simulink model "contrPUMA"  (R2026b)
settings: Solver=ode45  StopTime=7  MaxStep=1e-2  RelTol=1e-6  AbsTol=1e-8
libraries: slpidlib x3
settings Model: Creator=horia  LastModifiedBy=horia
settings DebuggingCC: AlgebraicLoopMsg=none

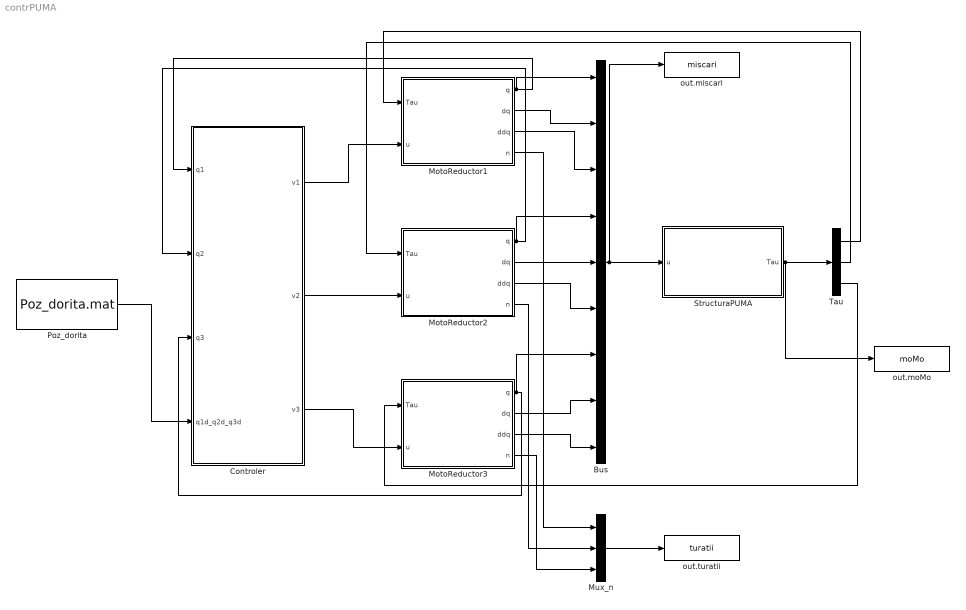
== system contrPUMA ==
  Bus : Mux  Inputs=9
  Controler : Subsystem
  MotoReductor1 : Subsystem
      settings: AttributesFormatString=RE 40 148867 + GP 52 C 230:1 (223101)
  MotoReductor2 : Subsystem
      settings: AttributesFormatString=RE 40 148867 + GP 52 C 230:1 (223101)
  MotoReductor3 : Subsystem
      settings: AttributesFormatString=RE 40 148867 + GP 42 C 74:1 (203123)
  Mux_n : Mux  Inputs=3
  Poz_dorita : FromFile  FileName=Poz_dorita.mat  SampleTime=0  ExtrapolationBeforeFirstDataPoint=Hold first value  ExtrapolationAfterLastDataPoint=Hold last value
  StructuraPUMA : Subsystem
  Tau : Demux  Outputs=3
  out.miscari : ToWorkspace  VariableName=miscari  SaveFormat=Timeseries  SampleTime=-1
  out.moMo : ToWorkspace  VariableName=moMo  SaveFormat=Timeseries  SampleTime=-1
  out.turatii : ToWorkspace  VariableName=turatii  SaveFormat=Timeseries  SampleTime=-1
  wires:
  Poz_dorita/1 -> Controler/4(q1d_q2d_q3d)
  Controler/1(v1) -> MotoReductor1/2(u)
  MotoReductor1/1(q) -> Controler/1(q1), Bus/1
  MotoReductor1/2(dq) -> Bus/2
  MotoReductor1/3(ddq) -> Bus/3
  MotoReductor1/4(n) -> Mux_n/1
  Tau/1 -> MotoReductor1/1(Tau)
  Controler/2(v2) -> MotoReductor2/2(u)
  MotoReductor2/1(q) -> Controler/2(q2), Bus/4
  MotoReductor2/2(dq) -> Bus/5
  MotoReductor2/3(ddq) -> Bus/6
  MotoReductor2/4(n) -> Mux_n/2
  Tau/2 -> MotoReductor2/1(Tau)
  Controler/3(v3) -> MotoReductor3/2(u)
  MotoReductor3/1(q) -> Controler/3(q3), Bus/7
  MotoReductor3/2(dq) -> Bus/8
  MotoReductor3/3(ddq) -> Bus/9
  MotoReductor3/4(n) -> Mux_n/3
  Tau/3 -> MotoReductor3/1(Tau)
  Bus/1 -> StructuraPUMA/1(u), out.miscari/1
  StructuraPUMA/1(Tau) -> Tau/1, out.moMo/1
  Mux_n/1 -> out.turatii/1

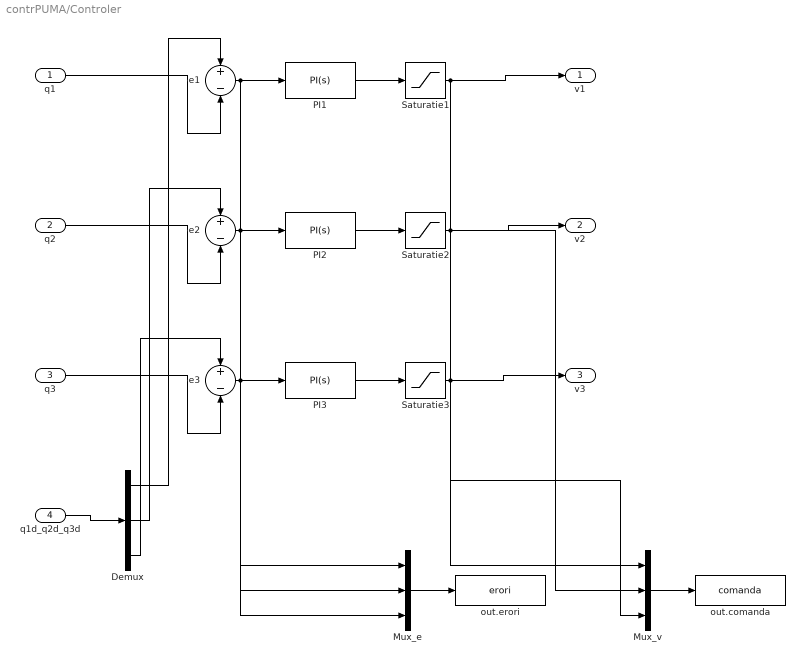
== system contrPUMA/Controler ==
  q1 : Inport  PortDimensions=1
  q2 : Inport  Port=2  PortDimensions=1
  q3 : Inport  Port=3  PortDimensions=1
  q1d_q2d_q3d : Inport  Port=4  PortDimensions=3
  Demux : Demux  Outputs=3
  Mux_e : Mux  Inputs=3
  Mux_v : Mux  Inputs=3
  PI1 : slpidlib/PID Controller  Controller=PI  Form=Parallel  TimeDomain=Continuous-time  UseExternalTs=off  SampleTime=-1  IntegratorMethod=Forward Euler  FilterMethod=Forward Euler  ControllerParametersSource=internal  P=108.8336797  I=567.4519736  UseKiTs=off  D=0  UseExternalDerivativeSource=off  N=100  UseFilter=on  TunerSelectOption=Transfer Function Based (PID Tuner App)  InitialConditionSource=internal  InitialConditionForIntegrator=0  InitialConditionForFilter=0  DifferentiatorICPrevScaledInput=0  ExternalReset=none  TrackingMode=off  Kt=1  LimitOutput=off  SatLimitsSource=internal  UpperSaturationLimit=inf  LowerSaturationLimit=-inf  LinearizeAsGain=on  AntiWindupMode=none  Kb=1  LimitIntegrator=off  UpperIntegratorSaturationLimit=inf  LowerIntegratorSaturationLimit=-inf  POutMin=[]  POutMax=[]  IOutMin=[]  IOutMax=[]  DOutMin=[]  DOutMax=[]  NOutMin=[]  NOutMax=[]  SumOutMin=[]  SumOutMax=[]  SaturationOutMin=[]  SaturationOutMax=[]  PParamMin=[]  PParamMax=[]  IParamMin=[]  IParamMax=[]  DParamMin=[]  DParamMax=[]  NParamMin=[]  NParamMax=[]  KbParamMin=[]  KbParamMax=[]  KtParamMin=[]  KtParamMax=[]  KbOutMin=[]  KbOutMax=[]  KtOutMin=[]  KtOutMax=[]  IntegratorOutMin=[]  IntegratorOutMax=[]  FilterOutMin=[]  FilterOutMax=[]  SumI1OutMin=[]  SumI1OutMax=[]  SumI2OutMin=[]  SumI2OutMax=[]  SumI3OutMin=[]  SumI3OutMax=[]  SumI4OutMin=[]  SumI4OutMax=[]  SumDOutMin=[]  SumDOutMax=[]  DifferentiatorOutMin=[]  DifferentiatorOutMax=[]  FilterDiffOutCoefMin=[]  FilterDiffOutCoefMax=[]  ReciprocalOutMin=[]  ReciprocalOutMax=[]  SumDenOutMin=[]  SumDenOutMax=[]  SumNumOutMin=[]  SumNumOutMax=[]  DivideOutMin=[]  DivideOutMax=[]  UdiffTsProdOutMin=[]  UdiffTsProdOutMax=[]  NTsProdOutMin=[]  NTsProdOutMax=[]  UintegralTsProdOutMin=[]  UintegralTsProdOutMax=[]  UngainTsProdOutMin=[]  UngainTsProdOutMax=[]  ClampingZeroOutDataTypeStr=Inherit: Inherit via back propagation  ClampingZeroOutMin=[]  ClampingZeroOutMax=[]  FilterDenConstantOutDataTypeStr=Inherit: Inherit via back propagation  FilterDenConstantOutMin=[]  FilterDenConstantOutMax=[]  PCopyOutDataTypeStr=Inherit: Inherit via back propagation  PCopyOutMin=[]  PCopyOutMax=[]  NCopyOutDataTypeStr=Inherit: Inherit via back propagation  NCopyOutMin=[]  NCopyOutMax=[]  IntegratorContinuousStateAttributes=''  IntegratorStateMustResolveToSignalObject=off  IntegratorRTWStateStorageClass=Auto  FilterContinuousStateAttributes=''  FilterStateMustResolveToSignalObject=off  FilterRTWStateStorageClass=Auto  ParallelPVariant=InternalParameters  IdealPVariant=Disabled  IVariant=InternalParameters  DVariant=Disabled  IntegratorVariant=Continuous  SatVariant=Disabled  AWVariant=Passthrough  PCopyVariant=Disabled  TRVariant=Disabled  FdbkBlocksVariant=Forward  IdealPFdbkVariant=Disabled  SatFdbkVariant=Disabled  DerivativeFilterVariant=Disabled  NVariant=Disabled  NCopyVariant=Disabled_SignalSpec  FilterICVariant=Disabled  IntegratorICVariant=InternalICs  ExternalResetVariant=Disabled  TRSumVariant=Passthrough  SumFdbkVariant=Disabled  SumVariant=Sum_PI  TsampFilterVariant=InternalTs  TsampNgainVariant=Passthrough  TsampIntegralVariant=Disabled_SignalSpec  ExternalSaturationOutDataTypeStr=Inherit: Same as second input  DerivativeSourceVariant=Disabled  PreIntVariant=InternalPreInt
  PI2 : slpidlib/PID Controller  Controller=PI  Form=Parallel  TimeDomain=Continuous-time  UseExternalTs=off  SampleTime=-1  IntegratorMethod=Forward Euler  FilterMethod=Forward Euler  ControllerParametersSource=internal  P=216.5960241  I=2247.519379  UseKiTs=off  D=0  UseExternalDerivativeSource=off  N=100  UseFilter=on  TunerSelectOption=Transfer Function Based (PID Tuner App)  InitialConditionSource=internal  InitialConditionForIntegrator=-1.121045947  InitialConditionForFilter=0  DifferentiatorICPrevScaledInput=0  ExternalReset=none  TrackingMode=off  Kt=1  LimitOutput=off  SatLimitsSource=internal  UpperSaturationLimit=inf  LowerSaturationLimit=-inf  LinearizeAsGain=on  AntiWindupMode=none  Kb=1  LimitIntegrator=off  UpperIntegratorSaturationLimit=inf  LowerIntegratorSaturationLimit=-inf  POutMin=[]  POutMax=[]  IOutMin=[]  IOutMax=[]  DOutMin=[]  DOutMax=[]  NOutMin=[]  NOutMax=[]  SumOutMin=[]  SumOutMax=[]  SaturationOutMin=[]  SaturationOutMax=[]  PParamMin=[]  PParamMax=[]  IParamMin=[]  IParamMax=[]  DParamMin=[]  DParamMax=[]  NParamMin=[]  NParamMax=[]  KbParamMin=[]  KbParamMax=[]  KtParamMin=[]  KtParamMax=[]  KbOutMin=[]  KbOutMax=[]  KtOutMin=[]  KtOutMax=[]  IntegratorOutMin=[]  IntegratorOutMax=[]  FilterOutMin=[]  FilterOutMax=[]  SumI1OutMin=[]  SumI1OutMax=[]  SumI2OutMin=[]  SumI2OutMax=[]  SumI3OutMin=[]  SumI3OutMax=[]  SumI4OutMin=[]  SumI4OutMax=[]  SumDOutMin=[]  SumDOutMax=[]  DifferentiatorOutMin=[]  DifferentiatorOutMax=[]  FilterDiffOutCoefMin=[]  FilterDiffOutCoefMax=[]  ReciprocalOutMin=[]  ReciprocalOutMax=[]  SumDenOutMin=[]  SumDenOutMax=[]  SumNumOutMin=[]  SumNumOutMax=[]  DivideOutMin=[]  DivideOutMax=[]  UdiffTsProdOutMin=[]  UdiffTsProdOutMax=[]  NTsProdOutMin=[]  NTsProdOutMax=[]  UintegralTsProdOutMin=[]  UintegralTsProdOutMax=[]  UngainTsProdOutMin=[]  UngainTsProdOutMax=[]  ClampingZeroOutDataTypeStr=Inherit: Inherit via back propagation  ClampingZeroOutMin=[]  ClampingZeroOutMax=[]  FilterDenConstantOutDataTypeStr=Inherit: Inherit via back propagation  FilterDenConstantOutMin=[]  FilterDenConstantOutMax=[]  PCopyOutDataTypeStr=Inherit: Inherit via back propagation  PCopyOutMin=[]  PCopyOutMax=[]  NCopyOutDataTypeStr=Inherit: Inherit via back propagation  NCopyOutMin=[]  NCopyOutMax=[]  IntegratorContinuousStateAttributes=''  IntegratorStateMustResolveToSignalObject=off  IntegratorRTWStateStorageClass=Auto  FilterContinuousStateAttributes=''  FilterStateMustResolveToSignalObject=off  FilterRTWStateStorageClass=Auto  ParallelPVariant=InternalParameters  IdealPVariant=Disabled  IVariant=InternalParameters  DVariant=Disabled  IntegratorVariant=Continuous  SatVariant=Disabled  AWVariant=Passthrough  PCopyVariant=Disabled  TRVariant=Disabled  FdbkBlocksVariant=Forward  IdealPFdbkVariant=Disabled  SatFdbkVariant=Disabled  DerivativeFilterVariant=Disabled  NVariant=Disabled  NCopyVariant=Disabled_SignalSpec  FilterICVariant=Disabled  IntegratorICVariant=InternalICs  ExternalResetVariant=Disabled  TRSumVariant=Passthrough  SumFdbkVariant=Disabled  SumVariant=Sum_PI  TsampFilterVariant=InternalTs  TsampNgainVariant=Passthrough  TsampIntegralVariant=Disabled_SignalSpec  ExternalSaturationOutDataTypeStr=Inherit: Same as second input  DerivativeSourceVariant=Disabled  PreIntVariant=InternalPreInt
  PI3 : slpidlib/PID Controller  Controller=PI  Form=Parallel  TimeDomain=Continuous-time  UseExternalTs=off  SampleTime=-1  IntegratorMethod=Forward Euler  FilterMethod=Forward Euler  ControllerParametersSource=internal  P=51.0415472  I=387.9236539  UseKiTs=off  D=0  UseExternalDerivativeSource=off  N=100  UseFilter=on  TunerSelectOption=Transfer Function Based (PID Tuner App)  InitialConditionSource=internal  InitialConditionForIntegrator=-0.5305099516  InitialConditionForFilter=0  DifferentiatorICPrevScaledInput=0  ExternalReset=none  TrackingMode=off  Kt=1  LimitOutput=off  SatLimitsSource=internal  UpperSaturationLimit=inf  LowerSaturationLimit=-inf  LinearizeAsGain=on  AntiWindupMode=none  Kb=1  LimitIntegrator=off  UpperIntegratorSaturationLimit=inf  LowerIntegratorSaturationLimit=-inf  POutMin=[]  POutMax=[]  IOutMin=[]  IOutMax=[]  DOutMin=[]  DOutMax=[]  NOutMin=[]  NOutMax=[]  SumOutMin=[]  SumOutMax=[]  SaturationOutMin=[]  SaturationOutMax=[]  PParamMin=[]  PParamMax=[]  IParamMin=[]  IParamMax=[]  DParamMin=[]  DParamMax=[]  NParamMin=[]  NParamMax=[]  KbParamMin=[]  KbParamMax=[]  KtParamMin=[]  KtParamMax=[]  KbOutMin=[]  KbOutMax=[]  KtOutMin=[]  KtOutMax=[]  IntegratorOutMin=[]  IntegratorOutMax=[]  FilterOutMin=[]  FilterOutMax=[]  SumI1OutMin=[]  SumI1OutMax=[]  SumI2OutMin=[]  SumI2OutMax=[]  SumI3OutMin=[]  SumI3OutMax=[]  SumI4OutMin=[]  SumI4OutMax=[]  SumDOutMin=[]  SumDOutMax=[]  DifferentiatorOutMin=[]  DifferentiatorOutMax=[]  FilterDiffOutCoefMin=[]  FilterDiffOutCoefMax=[]  ReciprocalOutMin=[]  ReciprocalOutMax=[]  SumDenOutMin=[]  SumDenOutMax=[]  SumNumOutMin=[]  SumNumOutMax=[]  DivideOutMin=[]  DivideOutMax=[]  UdiffTsProdOutMin=[]  UdiffTsProdOutMax=[]  NTsProdOutMin=[]  NTsProdOutMax=[]  UintegralTsProdOutMin=[]  UintegralTsProdOutMax=[]  UngainTsProdOutMin=[]  UngainTsProdOutMax=[]  ClampingZeroOutDataTypeStr=Inherit: Inherit via back propagation  ClampingZeroOutMin=[]  ClampingZeroOutMax=[]  FilterDenConstantOutDataTypeStr=Inherit: Inherit via back propagation  FilterDenConstantOutMin=[]  FilterDenConstantOutMax=[]  PCopyOutDataTypeStr=Inherit: Inherit via back propagation  PCopyOutMin=[]  PCopyOutMax=[]  NCopyOutDataTypeStr=Inherit: Inherit via back propagation  NCopyOutMin=[]  NCopyOutMax=[]  IntegratorContinuousStateAttributes=''  IntegratorStateMustResolveToSignalObject=off  IntegratorRTWStateStorageClass=Auto  FilterContinuousStateAttributes=''  FilterStateMustResolveToSignalObject=off  FilterRTWStateStorageClass=Auto  ParallelPVariant=InternalParameters  IdealPVariant=Disabled  IVariant=InternalParameters  DVariant=Disabled  IntegratorVariant=Continuous  SatVariant=Disabled  AWVariant=Passthrough  PCopyVariant=Disabled  TRVariant=Disabled  FdbkBlocksVariant=Forward  IdealPFdbkVariant=Disabled  SatFdbkVariant=Disabled  DerivativeFilterVariant=Disabled  NVariant=Disabled  NCopyVariant=Disabled_SignalSpec  FilterICVariant=Disabled  IntegratorICVariant=InternalICs  ExternalResetVariant=Disabled  TRSumVariant=Passthrough  SumFdbkVariant=Disabled  SumVariant=Sum_PI  TsampFilterVariant=InternalTs  TsampNgainVariant=Passthrough  TsampIntegralVariant=Disabled_SignalSpec  ExternalSaturationOutDataTypeStr=Inherit: Same as second input  DerivativeSourceVariant=Disabled  PreIntVariant=InternalPreInt
  Saturatie1 : Saturate  UpperLimit=24  LowerLimit=-24
  Saturatie2 : Saturate  UpperLimit=24  LowerLimit=-24
  Saturatie3 : Saturate  UpperLimit=24  LowerLimit=-24
  e1 : Sum  Inputs=+-
  e2 : Sum  Inputs=+-
  e3 : Sum  Inputs=+-
  out.comanda : ToWorkspace  VariableName=comanda  SaveFormat=Timeseries  SampleTime=-1
  out.erori : ToWorkspace  VariableName=erori  SaveFormat=Timeseries  SampleTime=-1
  v1 : Outport
  v2 : Outport  Port=2
  v3 : Outport  Port=3
  wires:
  q1d_q2d_q3d/1 -> Demux/1
  Demux/1 -> e1/1
  q1/1 -> e1/2
  e1/1 -> PI1/1, Mux_e/1
  PI1/1 -> Saturatie1/1
  Saturatie1/1 -> v1/1, Mux_v/1
  Demux/2 -> e2/1
  q2/1 -> e2/2
  e2/1 -> PI2/1, Mux_e/2
  PI2/1 -> Saturatie2/1
  Saturatie2/1 -> v2/1, Mux_v/2
  Demux/3 -> e3/1
  q3/1 -> e3/2
  e3/1 -> PI3/1, Mux_e/3
  PI3/1 -> Saturatie3/1
  Saturatie3/1 -> v3/1, Mux_v/3
  Mux_e/1 -> out.erori/1
  Mux_v/1 -> out.comanda/1

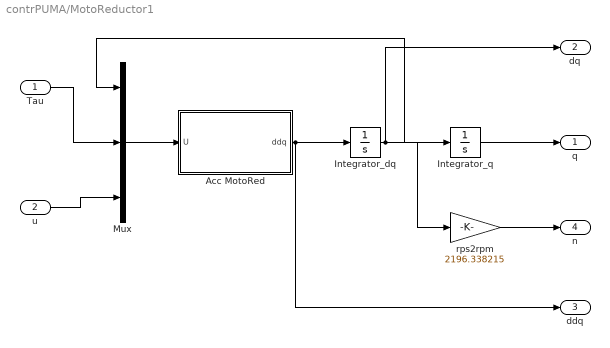
== system contrPUMA/MotoReductor1 ==
  Tau : Inport  PortDimensions=1
  u : Inport  Port=2  PortDimensions=1
  Acc MotoRed : MATLAB Function  TreatAsAtomicUnit=on
  Integrator_dq : Integrator
  Integrator_q : Integrator  InitialCondition=-0.4366271598
  Mux : Mux  Inputs=3
  rps2rpm : Gain  Gain=2196.338215
  q : Outport
  dq : Outport  Port=2
  ddq : Outport  Port=3
  n : Outport  Port=4
  wires:
  Integrator_dq/1 -> Mux/1, Integrator_q/1, dq/1, rps2rpm/1
  Tau/1 -> Mux/2
  u/1 -> Mux/3
  Mux/1 -> Acc MotoRed/1(U)
  Acc MotoRed/1(ddq) -> Integrator_dq/1, ddq/1
  Integrator_q/1 -> q/1
  rps2rpm/1 -> n/1

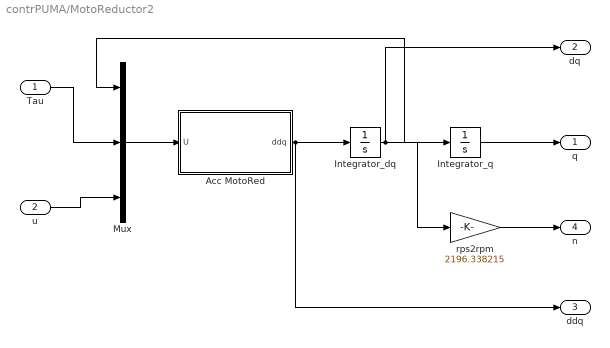
== system contrPUMA/MotoReductor2 ==
  Tau : Inport  PortDimensions=1
  u : Inport  Port=2  PortDimensions=1
  Acc MotoRed : MATLAB Function  TreatAsAtomicUnit=on
  Integrator_dq : Integrator
  Integrator_q : Integrator  InitialCondition=-0.5014914327
  Mux : Mux  Inputs=3
  rps2rpm : Gain  Gain=2196.338215
  q : Outport
  dq : Outport  Port=2
  ddq : Outport  Port=3
  n : Outport  Port=4
  wires:
  Integrator_dq/1 -> Mux/1, Integrator_q/1, dq/1, rps2rpm/1
  Tau/1 -> Mux/2
  u/1 -> Mux/3
  Mux/1 -> Acc MotoRed/1(U)
  Acc MotoRed/1(ddq) -> Integrator_dq/1, ddq/1
  Integrator_q/1 -> q/1
  rps2rpm/1 -> n/1

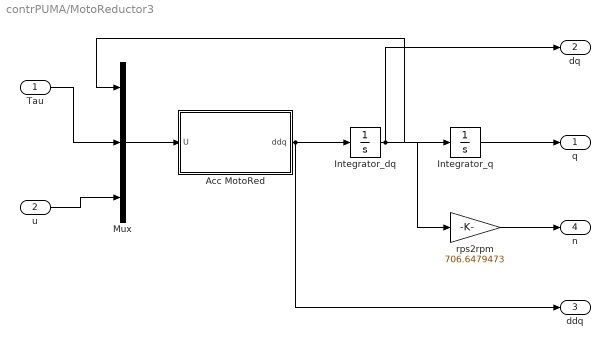
== system contrPUMA/MotoReductor3 ==
  Tau : Inport  PortDimensions=1
  u : Inport  Port=2  PortDimensions=1
  Acc MotoRed : MATLAB Function  TreatAsAtomicUnit=on
  Integrator_dq : Integrator
  Integrator_q : Integrator  InitialCondition=1.441639037
  Mux : Mux  Inputs=3
  rps2rpm : Gain  Gain=706.6479473
  q : Outport
  dq : Outport  Port=2
  ddq : Outport  Port=3
  n : Outport  Port=4
  wires:
  Integrator_dq/1 -> Mux/1, Integrator_q/1, dq/1, rps2rpm/1
  Tau/1 -> Mux/2
  u/1 -> Mux/3
  Mux/1 -> Acc MotoRed/1(U)
  Acc MotoRed/1(ddq) -> Integrator_dq/1, ddq/1
  Integrator_q/1 -> q/1
  rps2rpm/1 -> n/1

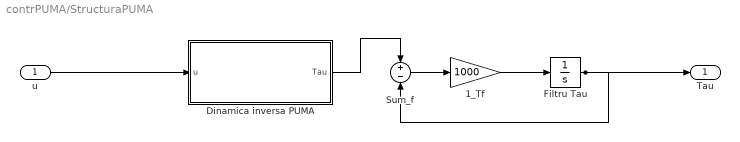
== system contrPUMA/StructuraPUMA ==
  u : Inport  PortDimensions=9
  1_Tf : Gain  Gain=1000
  Dinamica inversa PUMA : MATLAB Function  TreatAsAtomicUnit=on
  Filtru Tau : Integrator  InitialCondition=[0 -17.70907658 -2.854917126]
      settings: AttributesFormatString=Tf = 0.001 s
  Sum_f : Sum  Inputs=+-
  Tau : Outport
  wires:
  u/1 -> Dinamica inversa PUMA/1(u)
  Dinamica inversa PUMA/1(Tau) -> Sum_f/1
  Sum_f/1 -> 1_Tf/1
  1_Tf/1 -> Filtru Tau/1
  Filtru Tau/1 -> Sum_f/2, Tau/1

== matlab function contrPUMA/MotoReductor1/Acc MotoRed ==
  data: U input size=3; ddq output size=1
function ddq = acc_motored(U)
% Motor cc + reductor, cupla 1: RE 40 148867 + GP 52 C 230:1 (223101)
% U = [dq; tau; v]: viteza cuplei, cuplul cerut de structură, tensiunea
dq  = U(1);
tau = U(2);
v   = U(3);
% Parametrii motor + reductor (din Date_PUMA.m)
Ja  = 1.588e-05;   % inerția rotor + reductor [kg*m^2]
R   = 0.299;   % rezistența bobinajului [Ohm]
bm  = 5.21230339e-06;   % frecarea vâscoasă din motor [N*m*s/rad]
km  = 0.0302;   % constanta de cuplu [N*m/A]
ir  = 230;   % raportul de transmisie
ran = 0.68;   % randamentul reductorului
% Coeficienții
k1 = (bm + km^2/R)/Ja;   % dq
k2 = km/(Ja*ir*R);       % v
k3 = 1/(Ja*ran*ir^2);    % tau
% Ecuația
ddq = k2*v - k1*dq - k3*tau;
end

== matlab function contrPUMA/MotoReductor3/Acc MotoRed ==
  data: U input size=3; ddq output size=1
function ddq = acc_motored(U)
% Motor cc + reductor, cupla 3: RE 40 148867 + GP 42 C 74:1 (203123)
% U = [dq; tau; v]: viteza cuplei, cuplul cerut de structură, tensiunea
dq  = U(1);
tau = U(2);
v   = U(3);
% Parametrii motor + reductor (din Date_PUMA.m)
Ja  = 1.57e-05;   % inerția rotor + reductor [kg*m^2]
R   = 0.299;   % rezistența bobinajului [Ohm]
bm  = 5.21230339e-06;   % frecarea vâscoasă din motor [N*m*s/rad]
km  = 0.0302;   % constanta de cuplu [N*m/A]
ir  = 74;   % raportul de transmisie
ran = 0.72;   % randamentul reductorului
% Coeficienții
k1 = (bm + km^2/R)/Ja;   % dq
k2 = km/(Ja*ir*R);       % v
k3 = 1/(Ja*ran*ir^2);    % tau
% Ecuația
ddq = k2*v - k1*dq - k3*tau;
end

== matlab function contrPUMA/StructuraPUMA/Dinamica inversa PUMA ==
  data: u input size=9; Tau output size=3
function Tau = dinamica_inversa_PUMA(u)
% Modelul dinamic invers al structurii PUMA (Lagrange):
%   Tau = M(q)*ddq + C(q,dq)*dq + G(q) + Fv.*dq
% u = [q1 dq1 ddq1 q2 dq2 ddq2 q3 dq3 ddq3]
q   = [u(1); u(4); u(7)];
dq  = [u(2); u(5); u(8)];
ddq = [u(3); u(6); u(9)];
% Parametrii structurii (din Date_PUMA.m)
par.l1 = 0.4;  par.l2 = 0.2;  par.l3 = 0.3;  par.l4 = 0.4;  par.g = 9.81;
par.m2 = 3.053628059;  par.m3 = 2.790221044;  par.lc2 = 0.2;  par.lc3 = 0.1768795908;
par.I1zz = 0.06990899738;
par.I2 = [0.001374132627 0.0414021071 0.0414021071];   % [Ixx Iyy Izz] element 2
par.I3 = [0.00103059947 0.02692598826 0.02692598826];   % [Ixx Iyy Izz] element 3 + sarcina
Fv = [0 0 0]';  % frecarea vâscoasă în cuple
[M, C, G] = model_dinamic(q, dq, par);
Tau = M*ddq + C*dq + G + Fv.*dq;
end

function [M, C, G, V] = model_dinamic(q, dq, par)
% M(q)*ddq + C(q,dq)*dq + G(q) + Fv*dq = tau     (Lagrange)
%   r_c2 = l3 + lc2*c2,           z_c2 = l1 + l2 - lc2*s2
%   r_c3 = l3 + l4*c2 + lc3*c23,  z_c3 = l1 + l2 - l4*s2 - lc3*s23
%   w2 = [-s2*dq1; dq2; c2*dq1],  w3 = [-s23*dq1; dq2+dq3; c23*dq1]  (în axele proprii)
if nargin < 2 || isempty(dq), dq = [0; 0; 0]; end
l1 = par.l1; l2 = par.l2; l3 = par.l3; l4 = par.l4;
m2 = par.m2; m3 = par.m3; lc2 = par.lc2; lc3 = par.lc3; g = par.g;
I2xx = par.I2(1); I2yy = par.I2(2); I2zz = par.I2(3);
I3xx = par.I3(1); I3yy = par.I3(2); I3zz = par.I3(3);
s2 = sin(q(2)); c2 = cos(q(2)); s3 = sin(q(3)); c3 = cos(q(3));
s23 = sin(q(2)+q(3)); c23 = cos(q(2)+q(3));
dq1 = dq(1); dq2 = dq(2); dq3 = dq(3);

rc2 = l3 + lc2*c2;
rc3 = l3 + l4*c2 + lc3*c23;

% Matricea maselor
M11 = par.I1zz + I2xx*s2^2 + I2zz*c2^2 + I3xx*s23^2 + I3zz*c23^2 + m2*rc2^2 + m3*rc3^2;
M22 = I2yy + m2*lc2^2 + I3yy + m3*(l4^2 + lc3^2 + 2*l4*lc3*c3);
M23 = I3yy + m3*(lc3^2 + l4*lc3*c3);
M33 = I3yy + m3*lc3^2;
M = [M11 0   0;
     0   M22 M23;
     0   M23 M33];

% Matricea Coriolis/centrifugală (Christoffel)
% h2 = 1/2*dM11/dq2,  h3 = 1/2*dM11/dq3,  h = m3*l4*lc3*s3
h2 = (I2xx - I2zz)*s2*c2 + (I3xx - I3zz)*s23*c23 - m2*rc2*lc2*s2 - m3*rc3*(l4*s2 + lc3*s23);
h3 = (I3xx - I3zz)*s23*c23 - m3*rc3*lc3*s23;
h  = m3*l4*lc3*s3;
C = [ h2*dq2 + h3*dq3,  h2*dq1,   h3*dq1;
     -h2*dq1,          -h*dq3,   -h*(dq2 + dq3);
     -h3*dq1,           h*dq2,    0            ];

% Vectorul gravitațional G = dV/dq
G = [0;
     -g*(m2*lc2*c2 + m3*(l4*c2 + lc3*c23));
     -g*m3*lc3*c23];

% Energia potențială
V = g*(m2*(l1 + l2 - lc2*s2) + m3*(l1 + l2 - l4*s2 - lc3*s23));
end

== matlab function contrPUMA/MotoReductor2/Acc MotoRed ==
  data: U input size=3; ddq output size=1
function ddq = acc_motored(U)
% Motor cc + reductor, cupla 2: RE 40 148867 + GP 52 C 230:1 (223101)
% U = [dq; tau; v]: viteza cuplei, cuplul cerut de structură, tensiunea
dq  = U(1);
tau = U(2);
v   = U(3);
% Parametrii motor + reductor (din Date_PUMA.m)
Ja  = 1.588e-05;   % inerția rotor + reductor [kg*m^2]
R   = 0.299;   % rezistența bobinajului [Ohm]
bm  = 5.21230339e-06;   % frecarea vâscoasă din motor [N*m*s/rad]
km  = 0.0302;   % constanta de cuplu [N*m/A]
ir  = 230;   % raportul de transmisie
ran = 0.68;   % randamentul reductorului
% Coeficienții
k1 = (bm + km^2/R)/Ja;   % dq
k2 = km/(Ja*ir*R);       % v
k3 = 1/(Ja*ran*ir^2);    % tau
% Ecuația
ddq = k2*v - k1*dq - k3*tau;
end
